simulink model "Pseudo_Vector_Control"  (R2023a)
settings: Solver=FixedStepDiscrete  StartTime=0.0  StopTime=SC.T  FixedStep=P.dt  RelTol=1e-3
PreLoadFcn:
  | d_ = fileparts(get_param(bdroot,'FileName')); addpath(d_, fullfile(d_, '..', 'Common')); clear d_; pvc_init;
values from neighbouring files (symbols this model uses):
  DECIM = 10    [pvc_init.m]
  P = bldc_params()    [pvc_init.m]
  PVC = struct()    [pvc_init.m]
  TAB = struct()    [pvc_init.m]
undefined symbols (not defined in the file or in its folder): THETA_OFF
libraries: bldc_plant_lib x5, slpidlib x2, spspowerguiLib x1
settings Model: Creator=PC  LastModifiedBy=PC

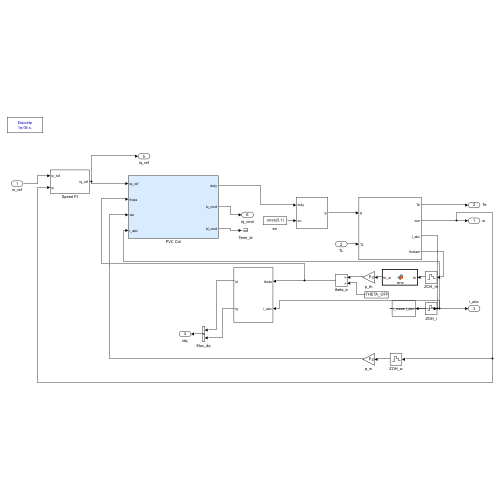
[thumbnail: Simulink's stored preview of the top-level diagram]
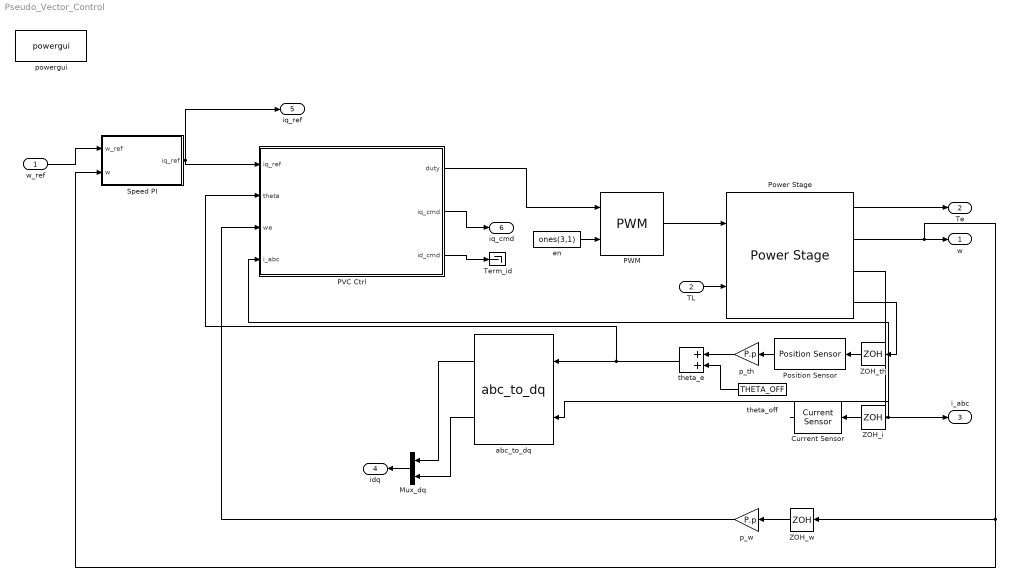
== system Pseudo_Vector_Control ==
  w_ref : Inport  Interpolate=off
  TL : Inport  Port=2  Interpolate=off
  Current Sensor : bldc_plant_lib/Current Sensor  Description=Phase-current sensors: i_meas = P.CS.M*(P.CS.gain.*i_abc + P.CS.off). Ideal by default (bldc_set_sensor).  SystemSampleTime=-1  VariantActivationTime=update diagram  Latency=0  AutoFrameSizeCalculation=off
  Mux_dq : Mux  Inputs=2
  PVC Ctrl : Subsystem
  PWM : bldc_plant_lib/PWM  SystemSampleTime=-1  VariantActivationTime=update diagram  Latency=0  AutoFrameSizeCalculation=off
  Position Sensor : bldc_plant_lib/Position Sensor  Description=Position sensor: quantized mechanical angle + mounting offset (P.ENC, bldc_set_encoder). Ideal by default.  SystemSampleTime=-1  VariantActivationTime=update diagram  Latency=0  AutoFrameSizeCalculation=off
      settings: LibrarySourceBlock=|
      | simulink/User-Defined
      | Functions/MATLAB Function
  Power Stage : bldc_plant_lib/Power Stage  SystemSampleTime=-1  VariantActivationTime=update diagram  Latency=0  AutoFrameSizeCalculation=off
  Speed PI : Subsystem
  Term_id : Terminator
  ZOH_i : ZeroOrderHold  SampleTime=P.Ts
  ZOH_th : ZeroOrderHold  SampleTime=P.Ts
  ZOH_w : ZeroOrderHold  SampleTime=P.Ts
  abc_to_dq : bldc_plant_lib/abc_to_dq  SystemSampleTime=-1  VariantActivationTime=update diagram  Latency=0  AutoFrameSizeCalculation=off
  en : Constant  Value=ones(3,1)
  p_th : Gain  Gain=P.p
  p_w : Gain  Gain=P.p
  powergui : spspowerguiLib/powergui  Priority=1  SimulationMode=Discrete  SampleTime=P.dt  frequency=60  Iterations=50  frequencyindice=0  Pbase=100e6  ErrMax=1e-4  UnitsV=kV  UnitsW=MW  buscounter=0  FunctionMessages=off  echomessages=off  EnableUseOfTLC=off  CurrentSourceSwitches=off  DisableSnubberDevices=off  DisableRonSwitches=off  DisableVfSwitches=off  DisplayEquations=off  AutomaticDiscreteSolvers=off  SolverType=Tustin/Backward Euler (TBE)  Interpol=off  ExternalGateDelay=off  methode=off  Ts=100  x0status=blocks  SPID=on  SwTol=0  HookPort=off  NonlinearTolerance=1e-4  nMaxIteration=100  ContinueOnMaxIteration=off  RestoreLinks=warning  ResistiveCurrentMeasurement=off  Frange=[0:2:500]  Ylog=off  Xlog=on  ShowGrid=off  save=off  variable=ZData  structure=0  ZoomFFT=off  StartTime=0.0  cycles=1  DisplayStyle=1  fundamental=60  FreqAxis=off  MaxFrequency=1000  frequencyindicesteady=1  RmsSteady=1  display=off
  theta_e : Sum
  theta_off : Constant  Value=THETA_OFF
  w : Outport  SampleTime=DECIM*P.dt
  Te : Outport  Port=2  SampleTime=DECIM*P.dt
  i_abc : Outport  Port=3  SampleTime=DECIM*P.dt
  idq : Outport  Port=4
  iq_ref : Outport  Port=5
  iq_cmd : Outport  Port=6
  wires:
  w_ref/1 -> Speed PI/1(w_ref)
  Speed PI/1(iq_ref) -> iq_ref/1, PVC Ctrl/1(iq_ref)
  TL/1 -> Power Stage/2
  PWM/1 -> Power Stage/1
  Power Stage/1 -> Te/1
  p_th/1 -> theta_e/1
  theta_off/1 -> theta_e/2
  ZOH_w/1 -> p_w/1
  abc_to_dq/1 -> Mux_dq/1
  abc_to_dq/2 -> Mux_dq/2
  Mux_dq/1 -> idq/1
  PVC Ctrl/1(duty) -> PWM/1
  PVC Ctrl/2(iq_cmd) -> iq_cmd/1
  PVC Ctrl/3(id_cmd) -> Term_id/1
  en/1 -> PWM/2
  Power Stage/2 -> ZOH_w/1, Speed PI/2(w), w/1
  Power Stage/3 -> i_abc/1, ZOH_i/1
  Power Stage/4 -> ZOH_th/1
  theta_e/1 -> abc_to_dq/1, PVC Ctrl/2(theta)
  p_w/1 -> PVC Ctrl/3(we)
  ZOH_i/1 -> Current Sensor/1
  Current Sensor/1 -> abc_to_dq/2, PVC Ctrl/4(i_abc)
  ZOH_th/1 -> Position Sensor/1
  Position Sensor/1 -> p_th/1

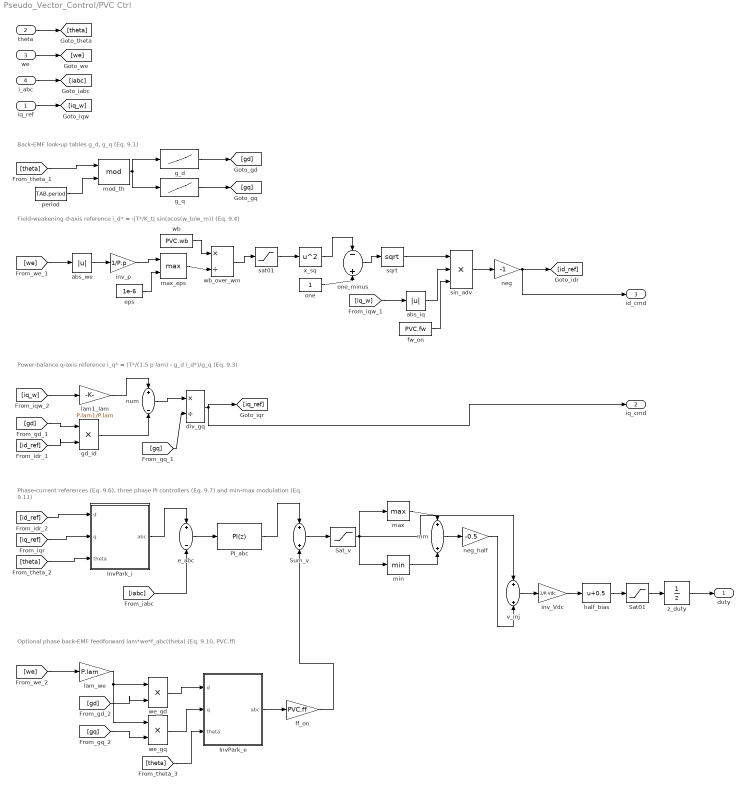
== system Pseudo_Vector_Control/PVC Ctrl ==
  note: Back-EMF look-up tables g_d, g_q (Eq. 9.1)
  note: Field-weakening d-axis reference i_d* = -|T*/K_t| sin(acos(w_b/w_m)) (Eq. 9.4)
  note: Power-balance q-axis reference i_q* = (T*/(1.5 p lam) - g_d i_d*)/g_q (Eq. 9.3)
  note: Phase-current references (Eq. 9.6), three phase PI controllers (Eq. 9.7) and min-max modulation (Eq. 9.11)
  note: Optional phase back-EMF feedforward lam*we*f_abc(theta) (Eq. 9.10, PVC.ff)
  iq_ref : Inport
  theta : Inport  Port=2
  we : Inport  Port=3
  i_abc : Inport  Port=4
  InvPark_e : Subsystem
  InvPark_i : Subsystem
  PI_abc : slpidlib/PID Controller  Controller=PI  Form=Parallel  TimeDomain=Discrete-time  UseExternalTs=off  SampleTime=P.Ts  IntegratorMethod=Forward Euler  FilterMethod=Forward Euler  ControllerParametersSource=internal  P=P.Kp_i  I=P.Ki_i  UseKiTs=off  D=0  N=100  UseFilter=on  TunerSelectOption=Transfer Function Based (PID Tuner App)  InitialConditionSource=internal  InitialConditionForIntegrator=0  InitialConditionForFilter=0  DifferentiatorICPrevScaledInput=0  ExternalReset=none  TrackingMode=off  Kt=1  LimitOutput=on  SatLimitsSource=internal  UpperSaturationLimit=P.Vm  LowerSaturationLimit=-P.Vm  LinearizeAsGain=on  AntiWindupMode=back-calculation  Kb=(P.Ki_i)/(P.Kp_i)  LimitIntegrator=off  UpperIntegratorSaturationLimit=inf  LowerIntegratorSaturationLimit=-inf  POutMin=[]  POutMax=[]  IOutMin=[]  IOutMax=[]  DOutMin=[]  DOutMax=[]  NOutMin=[]  NOutMax=[]  SumOutMin=[]  SumOutMax=[]  SaturationOutMin=[]  SaturationOutMax=[]  PParamMin=[]  PParamMax=[]  IParamMin=[]  IParamMax=[]  DParamMin=[]  DParamMax=[]  NParamMin=[]  NParamMax=[]  KbParamMin=[]  KbParamMax=[]  KtParamMin=[]  KtParamMax=[]  KbOutMin=[]  KbOutMax=[]  KtOutMin=[]  KtOutMax=[]  IntegratorOutMin=[]  IntegratorOutMax=[]  FilterOutMin=[]  FilterOutMax=[]  SumI1OutMin=[]  SumI1OutMax=[]  SumI2OutMin=[]  SumI2OutMax=[]  SumI3OutMin=[]  SumI3OutMax=[]  SumI4OutMin=[]  SumI4OutMax=[]  SumDOutMin=[]  SumDOutMax=[]  DifferentiatorOutMin=[]  DifferentiatorOutMax=[]  FilterDiffOutCoefMin=[]  FilterDiffOutCoefMax=[]  ReciprocalOutMin=[]  ReciprocalOutMax=[]  SumDenOutMin=[]  SumDenOutMax=[]  SumNumOutMin=[]  SumNumOutMax=[]  DivideOutMin=[]  DivideOutMax=[]  UdiffTsProdOutMin=[]  UdiffTsProdOutMax=[]  NTsProdOutMin=[]  NTsProdOutMax=[]  UintegralTsProdOutMin=[]  UintegralTsProdOutMax=[]  UngainTsProdOutMin=[]  UngainTsProdOutMax=[]  ClampingZeroOutDataTypeStr=Inherit: Inherit via back propagation  ClampingZeroOutMin=[]  ClampingZeroOutMax=[]  FilterDenConstantOutDataTypeStr=Inherit: Inherit via back propagation  FilterDenConstantOutMin=[]  FilterDenConstantOutMax=[]  PCopyOutDataTypeStr=Inherit: Inherit via back propagation  PCopyOutMin=[]  PCopyOutMax=[]  NCopyOutDataTypeStr=Inherit: Inherit via back propagation  NCopyOutMin=[]  NCopyOutMax=[]  IntegratorContinuousStateAttributes=''  IntegratorStateMustResolveToSignalObject=off  IntegratorRTWStateStorageClass=Auto  FilterContinuousStateAttributes=''  FilterStateMustResolveToSignalObject=off  FilterRTWStateStorageClass=Auto  ParallelPVariant=InternalParameters  IdealPVariant=Disabled  IVariant=InternalParameters  DVariant=Disabled  IntegratorVariant=Discrete  SatVariant=Enabled  AWVariant=BackCalculation  PCopyVariant=Disabled  TRVariant=Disabled  FdbkBlocksVariant=Forward  IdealPFdbkVariant=Disabled  SatFdbkVariant=Disabled  DerivativeFilterVariant=Disabled  NVariant=Disabled  NCopyVariant=Disabled_SignalSpec  FilterICVariant=Disabled  IntegratorICVariant=InternalICs  ExternalResetVariant=Disabled  TRSumVariant=Passthrough  SumFdbkVariant=Disabled  SumVariant=Sum_PI  TsampFilterVariant=InternalTs  TsampNgainVariant=Passthrough  TsampIntegralVariant=Disabled_SignalSpec  ExternalSaturationOutDataTypeStr=Inherit: Same as second input
  Sat01 : Saturate  UpperLimit=1  LowerLimit=0
  Sat_v : Saturate  UpperLimit=P.Vm  LowerLimit=-P.Vm
  Sum_v : Sum
  abs_iq : Abs
  abs_we : Abs
  div_gq : Product  Inputs=*/
  e_abc : Sum  Inputs=+-
  eps : Constant  Value=1e-6
  ff_on : Gain  Gain=PVC.ff
  fw_on : Constant  Value=PVC.fw
  g_d : Lookup_n-D  NumberOfTableDimensions=1  BreakpointsForDimension1=TAB.th  Table=TAB.gd  InternalRulePriority=Speed  RndMeth=Simplest
  g_q : Lookup_n-D  NumberOfTableDimensions=1  BreakpointsForDimension1=TAB.th  Table=TAB.gq  InternalRulePriority=Speed  RndMeth=Simplest
  gd_id : Product
  half_bias : Bias  Bias=0.5
  inv_Vdc : Gain  Gain=1/P.Vdc
  inv_p : Gain  Gain=1/P.p
  lam1_lam : Gain  Gain=P.lam1/P.lam
  lam_we : Gain  Gain=P.lam
  max : MinMax  Function=max
  max_eps : MinMax  Function=max  Inputs=2
  min : MinMax
  mm : Sum
  mod_th : Math  Operator=mod
  neg : Gain  Gain=-1
  neg_half : Gain  Gain=-0.5
  num : Sum  Inputs=+-
  one : Constant
  one_minus : Sum  Inputs=-+
  period : Constant  Value=TAB.period
  sat01 : Saturate  UpperLimit=1  LowerLimit=0
  sin_adv : Product  Inputs=3
  sqrt : Math  Operator=sqrt
  v_inj : Sum
  wb : Constant  Value=PVC.wb
  wb_over_wm : Product  Inputs=*/
  we_gd : Product
  we_gq : Product
  x_sq : Math  Operator=square
  z_duty : UnitDelay  InitialCondition=0.5*ones(3,1)  SampleTime=P.Ts
  duty : Outport
  iq_cmd : Outport  Port=2
  id_cmd : Outport  Port=3
  wires:
  theta/1 -> [theta]
  we/1 -> [we]
  i_abc/1 -> [iabc]
  iq_ref/1 -> [iq_w]
  [theta] -> mod_th/1
  period/1 -> mod_th/2
  mod_th/1 -> g_d/1, g_q/1
  g_d/1 -> [gd]
  g_q/1 -> [gq]
  [we] -> abs_we/1
  abs_we/1 -> inv_p/1
  inv_p/1 -> max_eps/1
  eps/1 -> max_eps/2
  wb/1 -> wb_over_wm/1
  max_eps/1 -> wb_over_wm/2
  wb_over_wm/1 -> sat01/1
  sat01/1 -> x_sq/1
  x_sq/1 -> one_minus/1
  one/1 -> one_minus/2
  one_minus/1 -> sqrt/1
  sqrt/1 -> sin_adv/1
  [iq_w] -> abs_iq/1
  abs_iq/1 -> sin_adv/2
  fw_on/1 -> sin_adv/3
  sin_adv/1 -> neg/1
  neg/1 -> [id_ref], id_cmd/1
  [iq_w] -> lam1_lam/1
  [gd] -> gd_id/1
  [id_ref] -> gd_id/2
  lam1_lam/1 -> num/1
  gd_id/1 -> num/2
  num/1 -> div_gq/1
  [gq] -> div_gq/2
  div_gq/1 -> [iq_ref], iq_cmd/1
  [id_ref] -> InvPark_i/1(d)
  [iq_ref] -> InvPark_i/2(q)
  [theta] -> InvPark_i/3(theta)
  InvPark_i/1(abc) -> e_abc/1
  [iabc] -> e_abc/2
  e_abc/1 -> PI_abc/1
  PI_abc/1 -> Sum_v/1
  Sum_v/1 -> Sat_v/1
  Sat_v/1 -> max/1, min/1, v_inj/1
  max/1 -> mm/1
  min/1 -> mm/2
  mm/1 -> neg_half/1
  neg_half/1 -> v_inj/2
  v_inj/1 -> inv_Vdc/1
  inv_Vdc/1 -> half_bias/1
  half_bias/1 -> Sat01/1
  Sat01/1 -> z_duty/1
  z_duty/1 -> duty/1
  [we] -> lam_we/1
  lam_we/1 -> we_gd/1, we_gq/1
  [gd] -> we_gd/2
  [gq] -> we_gq/2
  we_gd/1 -> InvPark_e/1(d)
  we_gq/1 -> InvPark_e/2(q)
  [theta] -> InvPark_e/3(theta)
  InvPark_e/1(abc) -> ff_on/1
  ff_on/1 -> Sum_v/2

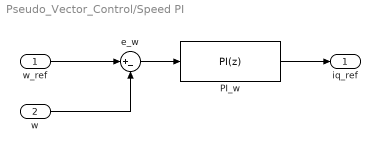
== system Pseudo_Vector_Control/Speed PI ==
  w_ref : Inport
  w : Inport  Port=2
  PI_w : slpidlib/PID Controller  Controller=PI  Form=Parallel  TimeDomain=Discrete-time  UseExternalTs=off  SampleTime=P.Tsw  IntegratorMethod=Forward Euler  FilterMethod=Forward Euler  ControllerParametersSource=internal  P=P.Kp_w_foc  I=P.Ki_w_foc  UseKiTs=off  D=0  N=100  UseFilter=on  TunerSelectOption=Transfer Function Based (PID Tuner App)  InitialConditionSource=internal  InitialConditionForIntegrator=0  InitialConditionForFilter=0  DifferentiatorICPrevScaledInput=0  ExternalReset=none  TrackingMode=off  Kt=1  LimitOutput=on  SatLimitsSource=internal  UpperSaturationLimit=P.Imax  LowerSaturationLimit=-P.Imax  LinearizeAsGain=off  AntiWindupMode=back-calculation  Kb=(P.Ki_w_foc)/(P.Kp_w_foc)  LimitIntegrator=off  UpperIntegratorSaturationLimit=inf  LowerIntegratorSaturationLimit=-inf  POutMin=[]  POutMax=[]  IOutMin=[]  IOutMax=[]  DOutMin=[]  DOutMax=[]  NOutMin=[]  NOutMax=[]  SumOutMin=[]  SumOutMax=[]  SaturationOutMin=[]  SaturationOutMax=[]  PParamMin=[]  PParamMax=[]  IParamMin=[]  IParamMax=[]  DParamMin=[]  DParamMax=[]  NParamMin=[]  NParamMax=[]  KbParamMin=[]  KbParamMax=[]  KtParamMin=[]  KtParamMax=[]  KbOutMin=[]  KbOutMax=[]  KtOutMin=[]  KtOutMax=[]  IntegratorOutMin=[]  IntegratorOutMax=[]  FilterOutMin=[]  FilterOutMax=[]  SumI1OutMin=[]  SumI1OutMax=[]  SumI2OutMin=[]  SumI2OutMax=[]  SumI3OutMin=[]  SumI3OutMax=[]  SumI4OutMin=[]  SumI4OutMax=[]  SumDOutMin=[]  SumDOutMax=[]  DifferentiatorOutMin=[]  DifferentiatorOutMax=[]  FilterDiffOutCoefMin=[]  FilterDiffOutCoefMax=[]  ReciprocalOutMin=[]  ReciprocalOutMax=[]  SumDenOutMin=[]  SumDenOutMax=[]  SumNumOutMin=[]  SumNumOutMax=[]  DivideOutMin=[]  DivideOutMax=[]  UdiffTsProdOutMin=[]  UdiffTsProdOutMax=[]  NTsProdOutMin=[]  NTsProdOutMax=[]  UintegralTsProdOutMin=[]  UintegralTsProdOutMax=[]  UngainTsProdOutMin=[]  UngainTsProdOutMax=[]  ClampingZeroOutDataTypeStr=Inherit: Inherit via back propagation  ClampingZeroOutMin=[]  ClampingZeroOutMax=[]  FilterDenConstantOutDataTypeStr=Inherit: Inherit via back propagation  FilterDenConstantOutMin=[]  FilterDenConstantOutMax=[]  PCopyOutDataTypeStr=Inherit: Inherit via back propagation  PCopyOutMin=[]  PCopyOutMax=[]  NCopyOutDataTypeStr=Inherit: Inherit via back propagation  NCopyOutMin=[]  NCopyOutMax=[]  IntegratorContinuousStateAttributes=''  IntegratorStateMustResolveToSignalObject=off  IntegratorRTWStateStorageClass=Auto  FilterContinuousStateAttributes=''  FilterStateMustResolveToSignalObject=off  FilterRTWStateStorageClass=Auto  ParallelPVariant=InternalParameters  IdealPVariant=Disabled  IVariant=InternalParameters  DVariant=Disabled  IntegratorVariant=Discrete  SatVariant=Enabled  AWVariant=BackCalculation  PCopyVariant=Disabled  TRVariant=Disabled  FdbkBlocksVariant=Forward  IdealPFdbkVariant=Disabled  SatFdbkVariant=Disabled  DerivativeFilterVariant=Disabled  NVariant=Disabled  NCopyVariant=Disabled_SignalSpec  FilterICVariant=Disabled  IntegratorICVariant=InternalICs  ExternalResetVariant=Disabled  TRSumVariant=Passthrough  SumFdbkVariant=Disabled  SumVariant=Sum_PI  TsampFilterVariant=InternalTs  TsampNgainVariant=Passthrough  TsampIntegralVariant=Disabled_SignalSpec  ExternalSaturationOutDataTypeStr=Inherit: Same as second input
      settings: LibrarySourceBlock=simulink/Discrete/Discrete PID Controller
  e_w : Sum  Inputs=|+-
  iq_ref : Outport
  wires:
  PI_w/1 -> iq_ref/1
  e_w/1 -> PI_w/1
  w/1 -> e_w/2
  w_ref/1 -> e_w/1

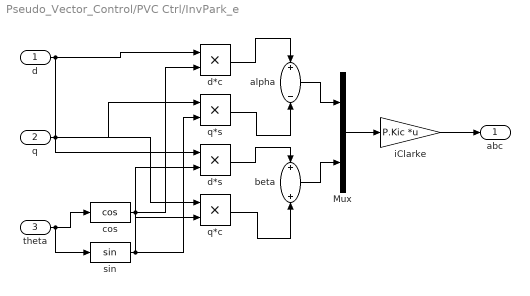
== system Pseudo_Vector_Control/PVC Ctrl/InvPark_e ==
  d : Inport
  q : Inport  Port=2
  theta : Inport  Port=3
  Mux : Mux  Inputs=2
  alpha : Sum  Inputs=+-
  beta : Sum
  cos : Trigonometry  Operator=cos
  d*c : Product
  d*s : Product
  iClarke : Gain  Gain=P.Kic  Multiplication=Matrix(K*u)
  q*c : Product
  q*s : Product
  sin : Trigonometry
  abc : Outport
  wires:
  iClarke/1 -> abc/1
  Mux/1 -> iClarke/1
  beta/1 -> Mux/2
  alpha/1 -> Mux/1
  q*c/1 -> beta/2
  d*s/1 -> beta/1
  q*s/1 -> alpha/2
  d*c/1 -> alpha/1
  sin/1 -> d*s/2, q*s/2
  q/1 -> q*c/1, q*s/1
  cos/1 -> q*c/2, d*c/2
  d/1 -> d*s/1, d*c/1
  theta/1 -> sin/1, cos/1

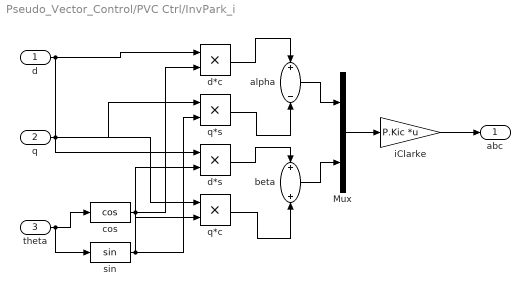
== system Pseudo_Vector_Control/PVC Ctrl/InvPark_i ==
  d : Inport
  q : Inport  Port=2
  theta : Inport  Port=3
  Mux : Mux  Inputs=2
  alpha : Sum  Inputs=+-
  beta : Sum
  cos : Trigonometry  Operator=cos
  d*c : Product
  d*s : Product
  iClarke : Gain  Gain=P.Kic  Multiplication=Matrix(K*u)
  q*c : Product
  q*s : Product
  sin : Trigonometry
  abc : Outport
  wires:
  theta/1 -> cos/1, sin/1
  d/1 -> d*c/1, d*s/1
  cos/1 -> d*c/2, q*c/2
  q/1 -> q*s/1, q*c/1
  sin/1 -> q*s/2, d*s/2
  d*c/1 -> alpha/1
  q*s/1 -> alpha/2
  d*s/1 -> beta/1
  q*c/1 -> beta/2
  alpha/1 -> Mux/1
  beta/1 -> Mux/2
  Mux/1 -> iClarke/1
  iClarke/1 -> abc/1
